simulink model "Palan_sim"  (R2022a)
settings: Solver=FixedStepDiscrete  StartTime=0.0  StopTime=inf  FixedStep=2e-4  RelTol=1e-3
PreLoadFcn:
  | waijung.modelPreload; % Required for working with Waijung Blockset. Do not remove.
values from neighbouring files (symbols this model uses):
  A = [   0   1    0   0 ... (first row only)    [ETAT_PAL_IDENT.m]    (also in Essai_boucle_ouverte.mat = [0 0 0 0 1 -7.87878787879 0 78.7878787879 0 0 0 -98.1 ... (1)
  C = [ 1 0 L 0]    [ETAT_PAL_IDENT.m]    (also in Essai_boucle_ouverte.mat = [1 0 0.1 0])
  x = [-0.000164031982422 -0.000155448913574 0 0.000431418418884 0.000983715057373 0.00135481357574 0.00139808654785 0.00121676921844 0.00107872486115 0.00114774703979 0.00138938426971 0.00161373615265 ... (7687 elements, 7687x1)]    [p1_cre_18V_droite_0m.mat]    (also in p1_cre_18V_droite_1m.mat = [0 8.61287117004e-06 0.000207126140594 0.000638604164124 0.0; p1_cre_18V_gauche_0m.mat = [0.00037956237793 0.000319242477417 0 -0.000526666641235 -0.; p1_cre_18V_gauche_1m.mat = [0 -8.58306884766e-06 -0.00020706653595 -0.000638604164124 -; p1_cre_24V_droite_0m.mat = [-0.000215768814087 -0.00020706653595 0 0.000604152679443 0.)
undefined symbols (not defined in the file or in its folder): CPHA_1Edge, CPOL_Low, disableTheCustomCode, DISTANCE_PER_TURN_X, Duplex, enableTheCustomCode, FirstBit_MSB, Full, HSEOSC, in1, initTheCustomCode, Link, LQFP64, modifySysTick, out1, outputCSHigh, outputCSLow, PPR_THETA, PPR_XY, PSC2V, ST, STM32F446RE, V2PSC, waitForPulse, xref
libraries: simulink x13, waijung_customcode x4, stm32f4_spi_lib x3, stm32f4_io_lib x2, stm32f4_device_config_lib x1
(part 2 of 2)

== matlab function Palan_sim/Castint16to2uint8_PWM_X ==
  data: x1 output; u input; x2 output
function [x1,x2]= castTo2uint8(u)
xy= typecast(u, 'uint8');
x1=xy(1);
x2=xy(2);
end

== matlab function Palan_sim/Button2PWM_Y ==
  data: K input; u input; y output
function y = Button2PWM(K,u)
%u i  the button output and is between -100 and  100, you have to mutiply
%it by 120 to obtain a value between -12000 and +12000, i.e., PMW
%admissible values
y = 120*u*int16(K);

== matlab function Palan_sim/Button2PWM_X ==
  data: K input; u input; y output
function y = Button2PWM(K,u)
%u i  the button output and is between -100 and  100, you have to mutiply
%it by 120 to obtain a value between -12000 and +12000, i.e., PMW
%admissible values
y = (120*u)*int16(K);
